simulink model "ASM_Traffic_MultiCore"  (R2026a)
settings: Solver=ode1  StartTime=SIM.tstart.v  StopTime=SIM.tend.v  FixedStep=SIM.StepSize.v
PostLoadFcn:
  | if any(exist('dsrtsu_mdlpostloadfcn', 'file') ~= 0), dsrtsu_mdlpostloadfcn('Execute', bdroot); end
  | try, asm_mdl_postloadfcn(bdroot, 'UpdateModel', 3600); catch, disp(lasterr); end,
InitFcn:
  | , if any(exist('rtifpga_mdlclblib', 'file') ~= 0), rtifpga_mdlclblib('Init', bdroot); end,
  | , if any(exist('dsmpb_private', 'file') ~= 0), dsmpb_private('dsmpb_mdlclblib', 'Init', bdroot); end,
model workspace (MAT data in the model file):
  asmReferencePath = [0 0.01 0.02 0.03 0.04 0.05 0.06 0.07 0.08 0.09 0.1 0.11 ... (350007 elements, 50001x7)]
  roadBounds : Simulink.Parameter (value not decoded)
  safetyAxes : Simulink.Parameter (value not decoded)
undefined symbols (not defined in the file): _to_, a0b2, ASM_BrakeHydraulics_DemoSystems, ASM_VehicleDynamics_DemoSystems, b98103fe8ad365046cd0, BrakeCircuit, controllerConfig, CPT, Crankshaft, DiscIntNeverNeededParam, dsmsi, FinalDriveAssembly, MDL, ModeSignals, mu, Pos_BrakePedal_Maneuver, rad, RefSignals, roadFamilyData, roadFamilyId, s_to_rpm, SIM, SoftECU, Suspension, Tire, Transmission
libraries: ASM_Traffic_lib x135, simulink x98, ASM_Utils_lib x77, ASM_VehicleDynamics_lib x70, ASM_Environment_lib x22, dsmpblib x20, dsmsilib x15, MDLD_Utils_lib x10, ASM_BrakeHydraulics_lib x3, sl_discontinuities x2
(part 3 of 65)

== system ASM_Traffic_MultiCore/AnimationInterface/Fellow_Doors ==
  Environment_Animation : Inport
  Bus Selector1 : BusSelector  OutputSignals=UserSignals_Customized.Fellow1_DoorFL,UserSignals_Customized.Fellow2_DoorFL,UserSignals_Customized.Fellow3_DoorFL,UserSignals_Customized.Fellow4_DoorFL,UserSignals_Customized.Fellow5_DoorFL,UserSignals_Customized.Fellow6_DoorFL,UserSignals_Customized.Fellow7_DoorFL,UserSignals_Customized.Fellow8_DoorFL,UserSignals_Customized.Fellow9_DoorFL,UserSignals_Customized.Fellow10_DoorFL,UserSignals_Customized.Fellow11_DoorFL,UserSignals_Customized.Fellow12_DoorFL,UserSignals_Customized.Fellow13_DoorFL,UserSignals_Customized.Fellow14_DoorFL,UserSignals_Customized.Fellow15_DoorFL,UserSignals_Customized.Fellow16_DoorFL,UserSignals_Customized.Fellow17_DoorFL,UserSignals_Customized.Fellow18_DoorFL,UserSignals_Customized.Fellow19_DoorFL,UserSignals_Customized.Fellow20_DoorFL,UserSignals_Customized.Fellow21_DoorFL,UserSignals_Customized.Fellow22_DoorFL,UserSignals_Customized.Fellow23_DoorFL,UserSignals_Customized.Fellow24_DoorFL,UserSignals_Customized.Fellow25_DoorFL,UserSignals_Customized.Fellow26_DoorFL,UserSignals_Customized.Fellow27_DoorFL,UserSignals_Customized.Fellow28_DoorFL,UserSignals_Customized.Fellow29_DoorFL,UserSignals_Customized.Fellow30_DoorFL  OutputAsBus=on
  Bus Selector2 : BusSelector  OutputSignals=UserSignals_Customized.Fellow1_DoorFR,UserSignals_Customized.Fellow2_DoorFR,UserSignals_Customized.Fellow3_DoorFR,UserSignals_Customized.Fellow4_DoorFR,UserSignals_Customized.Fellow5_DoorFR,UserSignals_Customized.Fellow6_DoorFR,UserSignals_Customized.Fellow7_DoorFR,UserSignals_Customized.Fellow8_DoorFR,UserSignals_Customized.Fellow9_DoorFR,UserSignals_Customized.Fellow10_DoorFR,UserSignals_Customized.Fellow11_DoorFR,UserSignals_Customized.Fellow12_DoorFR,UserSignals_Customized.Fellow13_DoorFR,UserSignals_Customized.Fellow14_DoorFR,UserSignals_Customized.Fellow15_DoorFR,UserSignals_Customized.Fellow16_DoorFR,UserSignals_Customized.Fellow17_DoorFR,UserSignals_Customized.Fellow18_DoorFR,UserSignals_Customized.Fellow19_DoorFR,UserSignals_Customized.Fellow20_DoorFR,UserSignals_Customized.Fellow21_DoorFR,UserSignals_Customized.Fellow22_DoorFR,UserSignals_Customized.Fellow23_DoorFR,UserSignals_Customized.Fellow24_DoorFR,UserSignals_Customized.Fellow25_DoorFR,UserSignals_Customized.Fellow26_DoorFR,UserSignals_Customized.Fellow27_DoorFR,UserSignals_Customized.Fellow28_DoorFR,UserSignals_Customized.Fellow29_DoorFR,UserSignals_Customized.Fellow30_DoorFR  OutputAsBus=on
  Bus Selector3 : BusSelector  OutputSignals=UserSignals_Customized.Fellow1_DoorRL,UserSignals_Customized.Fellow2_DoorRL,UserSignals_Customized.Fellow3_DoorRL,UserSignals_Customized.Fellow4_DoorRL,UserSignals_Customized.Fellow5_DoorRL,UserSignals_Customized.Fellow6_DoorRL,UserSignals_Customized.Fellow7_DoorRL,UserSignals_Customized.Fellow8_DoorRL,UserSignals_Customized.Fellow9_DoorRL,UserSignals_Customized.Fellow10_DoorRL,UserSignals_Customized.Fellow11_DoorRL,UserSignals_Customized.Fellow12_DoorRL,UserSignals_Customized.Fellow13_DoorRL,UserSignals_Customized.Fellow14_DoorRL,UserSignals_Customized.Fellow15_DoorRL,UserSignals_Customized.Fellow16_DoorRL,UserSignals_Customized.Fellow17_DoorRL,UserSignals_Customized.Fellow18_DoorRL,UserSignals_Customized.Fellow19_DoorRL,UserSignals_Customized.Fellow20_DoorRL,UserSignals_Customized.Fellow21_DoorRL,UserSignals_Customized.Fellow22_DoorRL,UserSignals_Customized.Fellow23_DoorRL,UserSignals_Customized.Fellow24_DoorRL,UserSignals_Customized.Fellow25_DoorRL,UserSignals_Customized.Fellow26_DoorRL,UserSignals_Customized.Fellow27_DoorRL,UserSignals_Customized.Fellow28_DoorRL,UserSignals_Customized.Fellow29_DoorRL,UserSignals_Customized.Fellow30_DoorRL  OutputAsBus=on
  Bus Selector4 : BusSelector  OutputSignals=UserSignals_Customized.Fellow1_DoorRR,UserSignals_Customized.Fellow2_DoorRR,UserSignals_Customized.Fellow3_DoorRR,UserSignals_Customized.Fellow4_DoorRR,UserSignals_Customized.Fellow5_DoorRR,UserSignals_Customized.Fellow6_DoorRR,UserSignals_Customized.Fellow7_DoorRR,UserSignals_Customized.Fellow8_DoorRR,UserSignals_Customized.Fellow9_DoorRR,UserSignals_Customized.Fellow10_DoorRR,UserSignals_Customized.Fellow11_DoorRR,UserSignals_Customized.Fellow12_DoorRR,UserSignals_Customized.Fellow13_DoorRR,UserSignals_Customized.Fellow14_DoorRR,UserSignals_Customized.Fellow15_DoorRR,UserSignals_Customized.Fellow16_DoorRR,UserSignals_Customized.Fellow17_DoorRR,UserSignals_Customized.Fellow18_DoorRR,UserSignals_Customized.Fellow19_DoorRR,UserSignals_Customized.Fellow20_DoorRR,UserSignals_Customized.Fellow21_DoorRR,UserSignals_Customized.Fellow22_DoorRR,UserSignals_Customized.Fellow23_DoorRR,UserSignals_Customized.Fellow24_DoorRR,UserSignals_Customized.Fellow25_DoorRR,UserSignals_Customized.Fellow26_DoorRR,UserSignals_Customized.Fellow27_DoorRR,UserSignals_Customized.Fellow28_DoorRR,UserSignals_Customized.Fellow29_DoorRR,UserSignals_Customized.Fellow30_DoorRR  OutputAsBus=on
  Bus Selector5 : BusSelector  OutputSignals=UserSignals_Customized.Fellow1_Hood,UserSignals_Customized.Fellow2_Hood,UserSignals_Customized.Fellow3_Hood,UserSignals_Customized.Fellow4_Hood,UserSignals_Customized.Fellow5_Hood,UserSignals_Customized.Fellow6_Hood,UserSignals_Customized.Fellow7_Hood,UserSignals_Customized.Fellow8_Hood,UserSignals_Customized.Fellow9_Hood,UserSignals_Customized.Fellow10_Hood,UserSignals_Customized.Fellow11_Hood,UserSignals_Customized.Fellow12_Hood,UserSignals_Customized.Fellow13_Hood,UserSignals_Customized.Fellow14_Hood,UserSignals_Customized.Fellow15_Hood,UserSignals_Customized.Fellow16_Hood,UserSignals_Customized.Fellow17_Hood,UserSignals_Customized.Fellow18_Hood,UserSignals_Customized.Fellow19_Hood,UserSignals_Customized.Fellow20_Hood,UserSignals_Customized.Fellow21_Hood,UserSignals_Customized.Fellow22_Hood,UserSignals_Customized.Fellow23_Hood,UserSignals_Customized.Fellow24_Hood,UserSignals_Customized.Fellow25_Hood,UserSignals_Customized.Fellow26_Hood,UserSignals_Customized.Fellow27_Hood,UserSignals_Customized.Fellow28_Hood,UserSignals_Customized.Fellow29_Hood,UserSignals_Customized.Fellow30_Hood  OutputAsBus=on
  Bus Selector6 : BusSelector  OutputSignals=UserSignals_Customized.Fellow1_Trunk,UserSignals_Customized.Fellow2_Trunk,UserSignals_Customized.Fellow3_Trunk,UserSignals_Customized.Fellow4_Trunk,UserSignals_Customized.Fellow5_Trunk,UserSignals_Customized.Fellow6_Trunk,UserSignals_Customized.Fellow7_Trunk,UserSignals_Customized.Fellow8_Trunk,UserSignals_Customized.Fellow9_Trunk,UserSignals_Customized.Fellow10_Trunk,UserSignals_Customized.Fellow11_Trunk,UserSignals_Customized.Fellow12_Trunk,UserSignals_Customized.Fellow13_Trunk,UserSignals_Customized.Fellow14_Trunk,UserSignals_Customized.Fellow15_Trunk,UserSignals_Customized.Fellow16_Trunk,UserSignals_Customized.Fellow17_Trunk,UserSignals_Customized.Fellow18_Trunk,UserSignals_Customized.Fellow19_Trunk,UserSignals_Customized.Fellow20_Trunk,UserSignals_Customized.Fellow21_Trunk,UserSignals_Customized.Fellow22_Trunk,UserSignals_Customized.Fellow23_Trunk,UserSignals_Customized.Fellow24_Trunk,UserSignals_Customized.Fellow25_Trunk,UserSignals_Customized.Fellow26_Trunk,UserSignals_Customized.Fellow27_Trunk,UserSignals_Customized.Fellow28_Trunk,UserSignals_Customized.Fellow29_Trunk,UserSignals_Customized.Fellow30_Trunk  OutputAsBus=on
  Bus to Vector{1..6} (6 alike) : BusToVector
  Data Type Conversion{1..6} (6 alike) : DataTypeConversion  OutDataTypeStr=double  SaturateOnIntegerOverflow=off  RndMeth=Floor
  Multiport Switch : MultiPortSwitch  Inputs=2  OutMin=30  OutMax=30  OutDataTypeStr=double  SaturateOnIntegerOverflow=off
  Multiport Switch{1..5} (5 alike) : MultiPortSwitch  Inputs=2  SaturateOnIntegerOverflow=off  InputSameDT=off
  Mux : Mux  Inputs=6
  Saturation : Saturate  UpperLimit=1  LowerLimit=0
  Select_Signals : Subsystem
  Fellow_Doors : Outport  VectorParamsAs1DForOutWhenUnconnected=off
  wires:
  Saturation/1 -> Fellow_Doors/1
  Environment_Animation/1 -> Select_Signals/1(Fellow_Doors), Bus Selector1/1, Bus Selector3/1, Bus Selector4/1, Bus Selector5/1, Bus Selector6/1, Bus Selector2/1
  Mux/1 -> Saturation/1
  Multiport Switch/1 -> Mux/1
  Multiport Switch1/1 -> Mux/2
  Multiport Switch2/1 -> Mux/3
  Multiport Switch3/1 -> Mux/4
  Multiport Switch5/1 -> Mux/6
  Multiport Switch4/1 -> Mux/5
  Select_Signals/7(SW_Trunk[Open0_1Closed]) -> Multiport Switch5/3
  Select_Signals/6(SW_Hood[Open0_1Closed]) -> Multiport Switch4/3
  Select_Signals/5(SW_DoorRR[Open0_1Closed]) -> Multiport Switch3/3
  Select_Signals/4(SW_DoorRL[Open0_1Closed]) -> Multiport Switch2/3
  Select_Signals/3(SW_DoorFR[Open0_1Closed]) -> Multiport Switch1/3
  Data Type Conversion2/1 -> Multiport Switch1/2
  Data Type Conversion3/1 -> Multiport Switch2/2
  Data Type Conversion4/1 -> Multiport Switch3/2
  Bus Selector6/1 -> Bus to Vector6/1
  Data Type Conversion6/1 -> Multiport Switch5/2
  Bus to Vector6/1 -> Data Type Conversion6/1
  Bus Selector5/1 -> Bus to Vector5/1
  Data Type Conversion5/1 -> Multiport Switch4/2
  Bus to Vector5/1 -> Data Type Conversion5/1
  Bus Selector4/1 -> Bus to Vector4/1
  Bus to Vector4/1 -> Data Type Conversion4/1
  Bus Selector3/1 -> Bus to Vector3/1
  Bus to Vector3/1 -> Data Type Conversion3/1
  Bus Selector2/1 -> Bus to Vector2/1
  Bus to Vector2/1 -> Data Type Conversion2/1
  Data Type Conversion1/1 -> Multiport Switch/2
  Bus to Vector1/1 -> Data Type Conversion1/1
  Bus Selector1/1 -> Bus to Vector1/1
  Select_Signals/2(SW_DoorFL[Open0_1Closed]) -> Multiport Switch/3
  Select_Signals/1(SW_ManualControl_Doors[1Scheduler|2Manual]) -> Multiport Switch/1, Multiport Switch1/1, Multiport Switch2/1, Multiport Switch3/1, Multiport Switch4/1, Multiport Switch5/1

== system ASM_Traffic_MultiCore/AnimationInterface/Fellow_Lights ==
  Environment_Animation : Inport
  Bus Selector : BusSelector  OutputSignals=Fellow1_TurnLights,Fellow2_TurnLights,Fellow3_TurnLights,Fellow4_TurnLights,Fellow5_TurnLights,Fellow6_TurnLights,Fellow7_TurnLights,Fellow8_TurnLights,Fellow9_TurnLights,Fellow10_TurnLights,Fellow11_TurnLights,Fellow12_TurnLights,Fellow13_TurnLights,Fellow14_TurnLights,Fellow15_TurnLights,Fellow16_TurnLights,Fellow17_TurnLights,Fellow18_TurnLights,Fellow19_TurnLights,Fellow20_TurnLights,Fellow21_TurnLights,Fellow22_TurnLights,Fellow23_TurnLights,Fellow24_TurnLights,Fellow25_TurnLights,Fellow26_TurnLights,Fellow27_TurnLights,Fellow28_TurnLights,Fellow29_TurnLights,Fellow30_TurnLights  OutputAsBus=on
  Bus Selector2 : BusSelector  OutputSignals=a_Fellows[m|s2],Settings,UserSignals_Customized
  Bus to Vector3 : BusToVector
  Coding : Subsystem
  Compare_Both : simulink/Logic and Bit Operations/Compare To Constant  relop===  const=3  OutDataTypeStr=boolean
  Compare_Turnlight_L : simulink/Logic and Bit Operations/Compare To Constant  relop===  const=1  OutDataTypeStr=boolean
  Compare_Turnlight_R : simulink/Logic and Bit Operations/Compare To Constant  relop===  const=2  OutDataTypeStr=boolean
  Gain : Gain  Gain=-1
  Multiport Switch : MultiPortSwitch  Inputs=2  SaturateOnIntegerOverflow=off  InputSameDT=off
  Multiport Switch4 : MultiPortSwitch  Inputs=2  SaturateOnIntegerOverflow=off  InputSameDT=off
  Mux : Mux  Inputs=3
  OR : Logic  Operator=OR  IconShape=distinctive  AllPortsSameDT=off  OutDataTypeStr=boolean
  OR1 : Logic  Operator=OR  IconShape=distinctive  AllPortsSameDT=off  OutDataTypeStr=boolean
  Relay : Relay  OnSwitchValue=1.3  OffSwitchValue=1.2  OutDataTypeStr=boolean
  Select_Signals : Subsystem
  TurnLights[0|1|2|3] : DataTypeConversion  OutDataTypeStr=uint32  SaturateOnIntegerOverflow=off  RndMeth=Floor
  Fellow_Light : Outport  VectorParamsAs1DForOutWhenUnconnected=off
  wires:
  Gain/1 -> Relay/1
  Bus Selector2/2 -> Select_Signals/1(Fellow_VehicleLights)  "<Settings>"
  Environment_Animation/1 -> Bus Selector2/1
  Select_Signals/3(SW_TurnLight[0Off|1Left|2Right|3Both]) -> Multiport Switch4/3
  Select_Signals/2(SW_BrakeLight[0Off|1On]) -> Multiport Switch/3
  Select_Signals/1(SW_ManualControl_Lights[1Scheduler|2Manual]) -> Multiport Switch/1, Multiport Switch4/1
  Bus to Vector3/1 -> TurnLights[0|1|2|3]/1
  Mux/1 -> Coding/1(FellowLights)
  Multiport Switch4/1 -> Compare_Both/1, Compare_Turnlight_R/1, Compare_Turnlight_L/1
  OR1/1 -> Mux/3
  OR/1 -> Mux/2
  Compare_Both/1 -> OR/2, OR1/2
  Multiport Switch/1 -> Mux/1
  Compare_Turnlight_R/1 -> OR1/1
  Compare_Turnlight_L/1 -> OR/1
  Relay/1 -> Multiport Switch/2
  TurnLights[0|1|2|3]/1 -> Multiport Switch4/2
  Coding/1(Out) -> Fellow_Light/1
  Bus Selector2/1 -> Gain/1  "<a_Fellows[m|s2]>"
  Bus Selector2/3 -> Bus Selector/1  "<UserSignals_Customized>"
  Bus Selector/1 -> Bus to Vector3/1

== system ASM_Traffic_MultiCore/AnimationInterface/OpenAnimationInterfaceModel ==

== system ASM_Traffic_MultiCore/AnimationInterface/Vehicle_Doors ==
  Environment_Animation : Inport
  Bus Selector : BusSelector  OutputSignals=Mnv_DoorFL[],Mnv_DoorFR[],Mnv_DoorRL[],Mnv_DoorRR[],Mnv_Hood[],Mnv_Trunk[]  OutputAsBus=on
  Bus Selector7 : BusSelector  OutputSignals=Sw_ManualControl_Doors[1Maneuver|2Manual]
  Bus Selector8 : BusSelector  OutputSignals=Sw_DoorFL[0Closed_1Open],Sw_DoorFR[0Closed_1Open],Sw_DoorRL[0Closed_1Open],Sw_DoorRR[0Closed_1Open],Sw_Hood[0Closed_1Open],Sw_Trunk[0Closed_1Open]  OutputAsBus=on
  Bus to Vector : BusToVector
  Bus to Vector7 : BusToVector
  Data Type Conversion : DataTypeConversion  OutDataTypeStr=double  SaturateOnIntegerOverflow=off  RndMeth=Floor
  Data Type Conversion7 : DataTypeConversion  OutDataTypeStr=uint32  SaturateOnIntegerOverflow=off  RndMeth=Floor
  Data Type Conversion8 : DataTypeConversion  OutDataTypeStr=double  SaturateOnIntegerOverflow=off  RndMeth=Floor
  Multiport Switch6 : MultiPortSwitch  Inputs=2  OutMin=30  OutMax=30  OutDataTypeStr=double  SaturateOnIntegerOverflow=off
  Saturation : Saturate  UpperLimit=1  LowerLimit=0
  ASM_Vehicle_Doors : Outport  VectorParamsAs1DForOutWhenUnconnected=off
  wires:
  Saturation/1 -> ASM_Vehicle_Doors/1
  Data Type Conversion7/1 -> Multiport Switch6/1
  Bus Selector7/1 -> Data Type Conversion7/1  "<Sw_ManualControl_Doors[1Maneuver|2Manual]>"
  Data Type Conversion8/1 -> Multiport Switch6/3
  Multiport Switch6/1 -> Saturation/1
  Bus to Vector7/1 -> Data Type Conversion8/1
  Bus to Vector/1 -> Data Type Conversion/1
  Bus Selector8/1 -> Bus to Vector7/1
  Data Type Conversion/1 -> Multiport Switch6/2
  Environment_Animation/1 -> Bus Selector/1, Bus Selector7/1, Bus Selector8/1
  Bus Selector/1 -> Bus to Vector/1

== system ASM_Traffic_MultiCore/AnimationInterface/Vehicle_Lights ==
  VehicleDynamics_Animation : Inport
  Environment_Animation : Inport  Port=2
  Bus Selector : BusSelector  OutputSignals=Sw_ManualControl_Lights[1Maneuver|2Manual],Sw_BrakeLight[0Off|1On],Sw_TurnLights[0Off|1Left|2Right|3Both],ASM_Vehicle_TurnLights[]
  Bus Selector13 : BusSelector  OutputSignals=p_Brake[FL;FR;RL;RR][bar]
  Cmp_BrakePres : simulink/Logic and Bit Operations/Compare To Constant  relop=>  const=3  OutDataTypeStr=boolean
  Coding : Subsystem
  Compare_Hazard : simulink/Logic and Bit Operations/Compare To Constant  relop===  const=3  OutDataTypeStr=boolean
  Compare_Turnlight_L : simulink/Logic and Bit Operations/Compare To Constant  relop===  const=1.0  OutDataTypeStr=boolean
  Compare_Turnlight_R : simulink/Logic and Bit Operations/Compare To Constant  relop===  const=2  OutDataTypeStr=boolean
  Data Type Conversion1 : DataTypeConversion  OutDataTypeStr=boolean  SaturateOnIntegerOverflow=off  RndMeth=Floor
  Data Type Conversion2 : DataTypeConversion  OutDataTypeStr=uint32  SaturateOnIntegerOverflow=off  RndMeth=Floor
  Data Type Conversion3 : DataTypeConversion  OutDataTypeStr=uint32  SaturateOnIntegerOverflow=off  RndMeth=Floor
  Data Type Conversion4 : DataTypeConversion  OutDataTypeStr=uint32  SaturateOnIntegerOverflow=off  RndMeth=Floor
  Gain : Gain  Gain=1/4
  Multiport Switch : MultiPortSwitch  Inputs=2  SaturateOnIntegerOverflow=off  InputSameDT=off
  Multiport Switch4 : MultiPortSwitch  Inputs=2  SaturateOnIntegerOverflow=off  InputSameDT=off
  Mux : Mux  Inputs=3
  OR : Logic  Operator=OR  IconShape=distinctive  AllPortsSameDT=off  OutDataTypeStr=boolean
  OR1 : Logic  Operator=OR  IconShape=distinctive  AllPortsSameDT=off  OutDataTypeStr=boolean
  Sum of Elements : Sum  Inputs=+
  ASM_Vehicle_Lights : Outport  VectorParamsAs1DForOutWhenUnconnected=off
  wires:
  Bus Selector13/1 -> Sum of Elements/1  "<p_Brake[FL;FR;RL;RR][bar]>"
  Compare_Turnlight_L/1 -> OR/1
  Gain/1 -> Cmp_BrakePres/1
  Multiport Switch/1 -> Mux/1
  Data Type Conversion3/1 -> Multiport Switch/1, Multiport Switch4/1
  Compare_Hazard/1 -> OR/2, OR1/2
  Bus Selector/1 -> Data Type Conversion3/1  "<Sw_ManualControl_Lights[1Maneuver|2Manual]>"
  Bus Selector/3 -> Data Type Conversion2/1  "<Sw_TurnLights[0Off|1Left|2Right|3Both]>"
  Data Type Conversion4/1 -> Multiport Switch4/2
  Sum of Elements/1 -> Gain/1
  Bus Selector/4 -> Data Type Conversion4/1  "<ASM_Vehicle_TurnLights[]>"
  Bus Selector/2 -> Data Type Conversion1/1  "<Sw_BrakeLight[0Off|1On]>"
  Compare_Turnlight_R/1 -> OR1/1
  OR1/1 -> Mux/3
  Cmp_BrakePres/1 -> Multiport Switch/2
  Data Type Conversion2/1 -> Multiport Switch4/3
  OR/1 -> Mux/2
  Data Type Conversion1/1 -> Multiport Switch/3
  Multiport Switch4/1 -> Compare_Hazard/1, Compare_Turnlight_R/1, Compare_Turnlight_L/1
  Mux/1 -> Coding/1(In)
  Coding/1(Out) -> ASM_Vehicle_Lights/1
  Environment_Animation/1 -> Bus Selector/1
  VehicleDynamics_Animation/1 -> Bus Selector13/1

== system ASM_Traffic_MultiCore/DomainControl/DriverAssistance ==
  note: Driver Assistance
  In : Inport
  Control : Subsystem
  Interface_In : Subsystem
  Interface_Out : Subsystem
  SignalInterface : Subsystem
  Out : Outport  VectorParamsAs1DForOutWhenUnconnected=off
  wires:
  In/1 -> Interface_In/1(In)
  Interface_In/1(Out) -> SignalInterface/1(In), Control/1(Interface_In)
  Interface_Out/1(Out) -> Out/1
  Control/1(Control) -> Interface_Out/1(In)

== system ASM_Traffic_MultiCore/DomainControl/StartSystem ==
  note: Start System
  In : Inport
  Control : Subsystem
  Interface_In : Subsystem
  Interface_Out : Subsystem
  SignalInterface : Subsystem
  Out : Outport  VectorParamsAs1DForOutWhenUnconnected=off
  wires:
  In/1 -> Interface_In/1(In)
  Interface_In/1(Out) -> SignalInterface/1(In), Control/1(Interface_In)
  Interface_Out/1(Out) -> Out/1
  Control/1(Control) -> Interface_Out/1(In)

== system ASM_Traffic_MultiCore/DomainControl/TorqueManager ==
  note: Torque Manager Basic
  In : Inport
  Control : Subsystem
  Interface_In : Subsystem
  Interface_Out : Subsystem
  SignalInterface : Subsystem
  Out : Outport  VectorParamsAs1DForOutWhenUnconnected=off
  wires:
  In/1 -> Interface_In/1(In)
  Control/1(Control) -> Interface_Out/1(In)
  Interface_In/1(Out) -> SignalInterface/1(In), Control/1(Interface_In)
  Interface_Out/1(Out) -> Out/1

== system ASM_Traffic_MultiCore/Driver/Interface_In ==
  note: Driver
  In : Inport
  Bus Creator1 : BusCreator  Inputs=1
  Bus Selector4 : BusSelector  OutputSignals=Environment.Plant.Sw_ModelPortBlocks[0Disabled|1Enabled],Environment.Plant.Sw_ModelDeskPlottingInterface[0Disabled|1Enabled],VehicleDynamics.Plant.v_x_Vehicle_CoG[km|h],VehicleDynamics.Plant.v_y_Vehicle_CoG[km|h],VehicleDynamics.Plant.Pos_x_Vehicle_CoorSys_E[m],VehicleDynamics.Plant.Pos_y_Vehicle_CoorSys_E[m],VehicleDynamics.Plant.Angle_Yaw_Vehicle_CoorSys_E[deg],VehicleDynamics.Plant.YawRate_Vehicle_CoG[deg|s],VehicleDynamics.Plant.m_TotalVehicle[kg],VehicleDynamics.Plant.F_Driving_Res[N],VehicleDynamics.Plant.Pos_x_CoG_Vehicle_Total[m],VehicleDynamics.Plant.Inertia_z_Vehicle_Total[kgm2],VehicleDynamics.Plant.CorneringStiffness_Tire_Front[N|rad],VehicleDynamics.Plant.CorneringStiffness_Tire_Rear[N|rad],VehicleDynamics.Plant.i_Steering_Mean[],Drivetrain.Plant.n_Engine[rpm],Drivetrain.Plant.omega_Out_Trm[rad|s],DomainControl.TorqueManager.Control.State_Engine[0|1|2|3|4],Environment.Plant.Reset_States[0|1],Environment.Plant.s_Vehicle_Init[m],Environment.Plant.Route_Direction_Init[],Environment.Plant.s_Total_Vehicle_Road[m],Environment.Plant.Curv_Preview_Road[1|m],Environment.Plant.Speed_Limit_Preview_Road[km|h],Environment.Plant.Pos_z_Preview_Road[m],Environment.Plant.Roll_Preview_Road[deg],Environment.Plant.Pitch_Preview_Road[deg],Environment.Plant.x_Preview_DriverCurv[m],Environment.Plant.y_Preview_DriverCurv[m],Environment.Plant.Pos_x_Preview_Road[m],Environment.Plant.Pos_y_Preview_Road[m],Environment.Plant.Dist_Border_Left[m],Environment.Plant.Dist_Border_Right[m],Environment.Plant.Curv_Vehicle_Road[1|m],Environment.Plant.Angle_Yaw_Veh_Road[deg],Environment.Plant.Pos_AccPedal_Maneuver[%],Environment.Plant.Pos_BrakePedal_Maneuver[%],Environment.Plant.Pos_ClutchPedal_Maneuver[%],Environment.Plant.Gear_Maneuver[],Environment.Plant.Angle_SteeringWheel_Maneuver[deg],Environment.Plant.SelectorLever_Maneuver[-3T|-2P|-1R|0N|1D],Environment.Plant.v_Vehicle_Ref_Maneuver[m|s],Environment.Plant.v_Vehicle_Preview_Ref_Maneuver[m|s],Environment.Plant.a_x_Max[m|s2],Environment.Plant.a_x_Min[m|s2],Environment.Plant.a_y_Max[m|s2],Environment.Plant.Gear_Max[0Off|1_n],Environment.Plant.a_x_Vehicle_Ref_TrafficDriver[m|s2],Environment.Plant.Width_Deadzone_LatCtrl[m],Environment.Plant.Pos_x_Ref_Vehicle_Road[m],Environment.Plant.Pos_y_Ref_Vehicle_Road[m],Environment.Plant.Enable_v_Init[0|1],Drivetrain.Plant.Mode_Transmission[1Manual|2Automatic],Environment.Plant.Mode_AcceleratorBrake[1Stim|2Driver],Environment.Plant.Mode_GearClutch[1Stim|2Driver|3OpenClutch|4RefGear],Environment.Plant.Mode_Steer[1Stim|2Driver|3Fix],Environment.Plant.Sw_LatDriver[1LatCtrl1|2LatCtrl2],Environment.Plant.Mode_LatCtrl[1Pos|2Yaw],Environment.Plant.Mode_AdaptVelocityToRoad[1Off|2On],Environment.Plant.Mode_ForceToRoad[1Off|2On],Environment.Plant.Mode_SelectorLever[1Stim|2Driver],Environment.Plant.Mode_CurvatureCalculation[1Road|2Driver],Environment.Plant.Mode_TrafficDriver[1Off|2On],Engine.Control.State_StartStop[1Off|2NotReady|3Ready|4EngStopped],Engine.Control.n_Engine_Idle_Set[rpm],Environment.Plant.Lane_ID_Vehicle[]
  ModelSignals : Subsystem
  Out : Outport  VectorParamsAs1DForOutWhenUnconnected=off
  wires:
  Bus Selector4/2 -> ModelSignals/2(Sw_ModelDeskPlottingInterface[0Disabled|1Enabled])  "<Sw_ModelDeskPlottingInterface[0Disabled|1Enabled]>"
  Bus Selector4/1 -> ModelSignals/1(Sw_ModelPortBlocks[0Disabled|1Enabled])  "<Sw_ModelPortBlocks[0Disabled|1Enabled]>"
  In/1 -> Bus Selector4/1
  Bus Selector4/51 -> ModelSignals/51(Pos_y_Ref_Vehicle_Road[m])  "<Pos_y_Ref_Vehicle_Road[m]>"
  Bus Selector4/50 -> ModelSignals/50(Pos_x_Ref_Vehicle_Road[m])  "<Pos_x_Ref_Vehicle_Road[m]>"
  Bus Selector4/49 -> ModelSignals/49(Width_Deadzone_LatCtrl[m])  "<Width_Deadzone_LatCtrl[m]>"
  Bus Selector4/48 -> ModelSignals/48(a_x_Vehicle_Ref_TrafficDriver[m|s2])  "<a_x_Vehicle_Ref_TrafficDriver[m|s2]>"
  Bus Selector4/47 -> ModelSignals/47(Gear_Max[0Off|1_n])  "<Gear_Max[0Off|1_n]>"
  Bus Selector4/46 -> ModelSignals/46(a_y_Max[m|s2])  "<a_y_Max[m|s2]>"
  Bus Selector4/45 -> ModelSignals/45(a_x_Min[m|s2])  "<a_x_Min[m|s2]>"
  Bus Selector4/44 -> ModelSignals/44(a_x_Max[m|s2])  "<a_x_Max[m|s2]>"
  Bus Selector4/43 -> ModelSignals/43(v_Vehicle_Preview_Ref_Maneuver[m|s])  "<v_Vehicle_Preview_Ref_Maneuver[m|s]>"
  Bus Selector4/42 -> ModelSignals/42(v_Vehicle_Ref_Maneuver[m|s])  "<v_Vehicle_Ref_Maneuver[m|s]>"
  Bus Selector4/41 -> ModelSignals/41(SelectorLever_Maneuver[-3T|-2P|-1R|0N|1D])  "<SelectorLever_Maneuver[-3T|-2P|-1R|0N|1D]>"
  Bus Selector4/40 -> ModelSignals/40(Angle_SteeringWheel_Maneuver[deg])  "<Angle_SteeringWheel_Maneuver[deg]>"
  Bus Selector4/39 -> ModelSignals/39(Gear_Maneuver[])  "<Gear_Maneuver[]>"
  Bus Selector4/38 -> ModelSignals/38(Pos_ClutchPedal_Maneuver[%])  "<Pos_ClutchPedal_Maneuver[%]>"
  Bus Selector4/37 -> ModelSignals/37(Pos_BrakePedal_Maneuver[%])  "<Pos_BrakePedal_Maneuver[%]>"
  Bus Selector4/36 -> ModelSignals/36(Pos_AccPedal_Maneuver[%])  "<Pos_AccPedal_Maneuver[%]>"
  Bus Selector4/35 -> ModelSignals/35(Angle_Yaw_Veh_Road[deg])  "<Angle_Yaw_Veh_Road[deg]>"
  Bus Selector4/34 -> ModelSignals/34(Curv_Veh_Road[1|m])  "<Curv_Vehicle_Road[1|m]>"
  Bus Selector4/33 -> ModelSignals/33(Dist_Border_Right[m])  "<Dist_Border_Right[m]>"
  Bus Selector4/32 -> ModelSignals/32(Dist_Border_Left[m])  "<Dist_Border_Left[m]>"
  Bus Selector4/31 -> ModelSignals/31(Pos_y_Preview_Road[m])  "<Pos_y_Preview_Road[m]>"
  Bus Selector4/30 -> ModelSignals/30(Pos_x_Preview_Road[m])  "<Pos_x_Preview_Road[m]>"
  Bus Selector4/29 -> ModelSignals/29(Pos_y_Preview_DriverCurv[m])  "<y_Preview_DriverCurv[m]>"
  Bus Selector4/28 -> ModelSignals/28(Pos_x_Preview_DriverCurv[m])  "<x_Preview_DriverCurv[m]>"
  Bus Selector4/27 -> ModelSignals/27(Pitch_Preview_Road[deg])  "<Pitch_Preview_Road[deg]>"
  Bus Selector4/26 -> ModelSignals/26(Roll_Preview_Road[deg])  "<Roll_Preview_Road[deg]>"
  Bus Selector4/25 -> ModelSignals/25(Pos_z_Preview_Road[m])  "<Pos_z_Preview_Road[m]>"
  Bus Selector4/24 -> ModelSignals/24(Speed_Limit_Preview_Road[km|h])  "<Speed_Limit_Preview_Road[km|h]>"
  Bus Selector4/23 -> ModelSignals/23(Curv_Preview_Road[1|m])  "<Curv_Preview_Road[1|m]>"
  Bus Selector4/22 -> ModelSignals/22(s_Total_Vehicle_Road[m])  "<s_Total_Vehicle_Road[m]>"
  Bus Selector4/21 -> ModelSignals/21(Route_Direction_Init[])  "<Route_Direction_Init[]>"
  Bus Selector4/20 -> ModelSignals/20(s_Vehicle_Init[m])  "<s_Vehicle_Init[m]>"
  Bus Selector4/19 -> ModelSignals/19(Reset_States[0|1])  "<Reset_States[0|1]>"
  Bus Creator1/1 -> Out/1
  Bus Selector4/52 -> ModelSignals/52(Enable_v_Init[0|1])  "<Enable_v_Init[0|1]>"
  Bus Selector4/53 -> ModelSignals/53(Mode_Transmission[1Manual|2Automatic])  "<Mode_Transmission[1Manual|2Automatic]>"
  Bus Selector4/54 -> ModelSignals/54(Mode_AcceleratorBrake[1Stim|2Driver])  "<Mode_AcceleratorBrake[1Stim|2Driver]>"
  Bus Selector4/55 -> ModelSignals/55(Mode_GearClutch[1Stim|2Driver|3OpenClutch|4RefGear])  "<Mode_GearClutch[1Stim|2Driver|3OpenClutch|4RefGear]>"
  Bus Selector4/56 -> ModelSignals/56(Mode_Steer[1Stim|2Driver|3Fix])  "<Mode_Steer[1Stim|2Driver|3Fix]>"
  Bus Selector4/57 -> ModelSignals/57(Sw_LatDriver[1LatCtrl1|2LatCtrl2])  "<Sw_LatDriver[1LatCtrl1|2LatCtrl2]>"
  Bus Selector4/58 -> ModelSignals/58(Mode_LatCtrl[1Pos|2Yaw])  "<Mode_LatCtrl[1Pos|2Yaw]>"
  Bus Selector4/59 -> ModelSignals/59(Mode_AdaptVelocityToRoad[1Off|2On])  "<Mode_AdaptVelocityToRoad[1Off|2On]>"
  Bus Selector4/60 -> ModelSignals/60(Mode_ForceToRoad[1Off|2On])  "<Mode_ForceToRoad[1Off|2On]>"
  Bus Selector4/61 -> ModelSignals/61(Mode_SelectorLever[1Stim|2Driver])  "<Mode_SelectorLever[1Stim|2Driver]>"
  Bus Selector4/62 -> ModelSignals/62(Mode_CurvatureCalculation[1Road|2Driver])  "<Mode_CurvatureCalculation[1Road|2Driver]>"
  Bus Selector4/63 -> ModelSignals/63(Mode_TrafficDriver[1Off|2On])  "<Mode_TrafficDriver[1Off|2On]>"
  Bus Selector4/65 -> ModelSignals/65(n_Engine_Idle_Set[rpm])  "<n_Engine_Idle_Set[rpm]>"
  Bus Selector4/64 -> ModelSignals/64(State_StartStop[1Off|2NotReady|3Ready|4EngStopped])  "<State_StartStop[1Off|2NotReady|3Ready|4EngStopped]>"
  Bus Selector4/18 -> ModelSignals/18(State_Engine[0|1|2|3|4])  "<State_Engine[0|1|2|3|4]>"
  Bus Selector4/17 -> ModelSignals/17(omega_Out_Trm[rad|s])  "<omega_Out_Trm[rad|s]>"
  Bus Selector4/16 -> ModelSignals/16(n_Engine[rpm])  "<n_Engine[rpm]>"
  Bus Selector4/15 -> ModelSignals/15(i_Steering_Mean[])  "<i_Steering_Mean[]>"
  Bus Selector4/14 -> ModelSignals/14(CorneringStiffness_Tire_Rear[N|rad])  "<CorneringStiffness_Tire_Rear[N|rad]>"
  Bus Selector4/13 -> ModelSignals/13(CorneringStiffness_Tire_Front[N|rad])  "<CorneringStiffness_Tire_Front[N|rad]>"
  Bus Selector4/12 -> ModelSignals/12(Inertia_z_Vehicle_Total[kgm2])  "<Inertia_z_Vehicle_Total[kgm2]>"
  Bus Selector4/11 -> ModelSignals/11(Pos_x_CoG_Vehicle_Total[m])  "<Pos_x_CoG_Vehicle_Total[m]>"
  Bus Selector4/10 -> ModelSignals/10(F_Driving_Res[N])  "<F_Driving_Res[N]>"
  Bus Selector4/9 -> ModelSignals/9(m_Total_Vehicle[kg])  "<m_TotalVehicle[kg]>"
  Bus Selector4/8 -> ModelSignals/8(YawRate_Vehicle[deg|s])  "<YawRate_Vehicle_CoG[deg|s]>"
  Bus Selector4/7 -> ModelSignals/7(Angle_Yaw_Vehicle_CoorSys_E[deg])  "<Angle_Yaw_Vehicle_CoorSys_E[deg]>"
  Bus Selector4/6 -> ModelSignals/6(Pos_y_Vehicle_CoorSys_E[m])  "<Pos_y_Vehicle_CoorSys_E[m]>"
  Bus Selector4/5 -> ModelSignals/5(Pos_x_Vehicle_CoorSys_E[m])  "<Pos_x_Vehicle_CoorSys_E[m]>"
  Bus Selector4/4 -> ModelSignals/4(v_y_Vehicle_CoG[km|h])  "<v_y_Vehicle_CoG[km|h]>"
  Bus Selector4/3 -> ModelSignals/3(v_x_Vehicle_CoG[km|h])  "<v_x_Vehicle_CoG[km|h]>"
  ModelSignals/1(Out) -> Bus Creator1/1
  Bus Selector4/66 -> ModelSignals/66(Lane_ID_Vehicle[])  "<Lane_ID_Vehicle[]>"

== system ASM_Traffic_MultiCore/Driver/Interface_Out ==
  note: Driver
  In : Inport
  Bus Creator1 : BusCreator  Inputs=1
  Bus Selector2 : BusSelector  OutputSignals=OutputSignals.Pos_AccPedal[%],OutputSignals.Pos_BrakePedal[%],OutputSignals.Pos_ClutchPedal[%],OutputSignals.Gear[],OutputSignals.SelectorLever[-3T|-2P|-1R|0N|1D],OutputSignals.s_Preview[m],OutputSignals.Angle_SteeringWheel[deg],LongitudinalController.LongCtrl.t_Preview[s]
  Plant_ModelSignals : Subsystem
  Out : Outport  VectorParamsAs1DForOutWhenUnconnected=off
  wires:
  Bus Selector2/6 -> Plant_ModelSignals/6(s_Preview[m])  "<s_Preview[m]>"
  Bus Selector2/8 -> Plant_ModelSignals/8(t_Preview_vRef_Driver[s])  "<t_Preview[s]>"
  Bus Selector2/5 -> Plant_ModelSignals/5(SelectorLever[-3T|-2P|-1R|0N|1D])  "<SelectorLever[-3T|-2P|-1R|0N|1D]>"
  Bus Selector2/4 -> Plant_ModelSignals/4(Gear[])  "<Gear[]>"
  Bus Selector2/3 -> Plant_ModelSignals/3(Pos_ClutchPedal[%])  "<Pos_ClutchPedal[%]>"
  Bus Selector2/2 -> Plant_ModelSignals/2(Pos_BrakePedal[%])  "<Pos_BrakePedal[%]>"
  Bus Selector2/1 -> Plant_ModelSignals/1(Pos_AccPedal[%])  "<Pos_AccPedal[%]>"
  In/1 -> Bus Selector2/1
  Bus Selector2/7 -> Plant_ModelSignals/7(Angle_SteeringWheel[deg])  "<Angle_SteeringWheel[deg]>"
  Bus Creator1/1 -> Out/1  "Driver"
  Plant_ModelSignals/1(Out) -> Bus Creator1/1

== system ASM_Traffic_MultiCore/Driver/Plant ==
  note: Driver
  Interface_In : Inport
  steering_wheel[deg] : Inport  Port=2
  Driver : Subsystem
  UserInterface : Subsystem
  Plant : Outport  VectorParamsAs1DForOutWhenUnconnected=off
  wires:
  Driver/1(ASMSignalBus) -> Plant/1, UserInterface/1(In)
  Interface_In/1 -> Driver/2(Interface_In), UserInterface/2(Interface_In)
  UserInterface/1(Out) -> Driver/1(UserInterface)
  steering_wheel[deg]/1 -> Driver/3(steering_wheel[deg])

== system ASM_Traffic_MultiCore/Driver/SignalInterface ==
  In : Inport
  ASMSignalInterface : Subsystem  mask(ASM_SIGNAL_INTERFACE){LabelTextfield=Driver}
      mask prompts: LabelTextfield "Label"
      mask help:
      | The ASMSignalInterface block processes the ASMSignalBus and provides a vector-based interface for each signal (e.g. ModelDesk Plotting).
      |
      | Always push the update button after you have changed the signal bus structure in order to synchronize the signal interface. The update may take a few seconds.
      | A modified model must be reloaded in ModelDesk to keep consistency of ModelDesk and simulation model plot signals. Therefore select ''Update Model'' from the ''Simulation Model'' context menu of the ModelDesk Project Navigator.
      settings: AttributesFormatString=Label: %<LabelTextfield>
      settings: CopyFcn=|
      | try
      |  set_param(gcb,'LinkStatus', 'none')
      | catch
      | end
      mask Help: eval(['asm_modelhelp(gcbh,''tool'',''ASM_Utils_lib'', ''ASMSIGNALINTERFACE'')'])
      mask DialogControl Hint Prompt: For changes of Label first apply change and then push "Update".
      mask DialogControl UpdateButton Prompt: Update
      mask DialogControl UpdateButton Callback: asm_mdld_plot_block_update(bdroot(gcb), 'update', 'current');
      mask DialogControl UpdateAllButton Prompt: Update All
      mask DialogControl UpdateAllButton Callback: asm_mdld_plot_block_update(bdroot(gcb), 'update', 'all');
  Bus Selector Disable Signals : BusSelector  OutputSignals=ExternalModel.Sw_ModelPortBlocks[0Disabled|1Enabled],ExternalModel.Sw_ModelDeskPlottingInterface[0Disabled|1Enabled]
  ExternalOutports : Subsystem  TreatAsAtomicUnit=on
  wires:
  Bus Selector Disable Signals/2 -> ASMSignalInterface/Enable  "<Sw_ModelDeskPlottingInterface[0Disabled|1Enabled]>"
  Bus Selector Disable Signals/1 -> ExternalOutports/Enable  "<Sw_ModelPortBlocks[0Disabled|1Enabled]>"
  In/1 -> Bus Selector Disable Signals/1
  [ASMBUS_Driver_Plant] -> ASMSignalInterface/1(ASMSignalBus), ExternalOutports/1(In1)

== system ASM_Traffic_MultiCore/Drivetrain/Control ==
  note: Drivetrain Control
  Interface_In : Inport
  Plant : Inport  Port=2
  SoftECU_Drivetrain : Subsystem
  Sw_ECU_Signals : Subsystem
  UserInterface : Subsystem
  Control : Outport  VectorParamsAs1DForOutWhenUnconnected=off
  wires:
  Interface_In/1 -> SoftECU_Drivetrain/2(Interface_In), Sw_ECU_Signals/2(ExternalECU)
  SoftECU_Drivetrain/2(Out) -> Sw_ECU_Signals/1(SoftECU)
  Sw_ECU_Signals/1(ECU_Signals) -> Control/1
  SoftECU_Drivetrain/1(ASMSignalBus) -> UserInterface/1(In)
  UserInterface/1(Out) -> SoftECU_Drivetrain/1(UserInterface)
  Plant/1 -> SoftECU_Drivetrain/3(Plant)

== system ASM_Traffic_MultiCore/Drivetrain/Interface_In ==
  note: Drivetrain
  In : Inport
  Bus Creator1 : BusCreator  Inputs=2
  Bus Selector5 : BusSelector  OutputSignals=Environment.Plant.Sw_ModelPortBlocks[0Disabled|1Enabled],Environment.Plant.Sw_ModelDeskPlottingInterface[0Disabled|1Enabled],Environment.Plant.n_Engine_Set[rpm],Environment.Plant.Sw_Testbench[0Off|1On],Driver.Plant.Pos_ClutchPedal[%],Driver.Plant.Gear[],Environment.Plant.Reset_States[0|1],Engine.Plant.Trq_MeanEff_Engine[Nm],VehicleDynamics.Plant.omega_Wheel[FL;FR;RL;RR][rad|s],Environment.Plant.Enable_v_Init[0|1],Driver.Plant.Pos_AccPedal[%],Driver.Plant.SelectorLever[-3T|-2P|-1R|0N|1D],Environment.Plant.Sw_TipShift_Maneuver[-1Down|0Off|1Up],Environment.Plant.Gear_Maneuver[],Environment.Plant.Mode_GearClutch[1Stim|2Driver|3OpenClutch|4RefGear],Environment.Plant.Gear_Max[0Off|1_n],DomainControl.TorqueManager.Control.State_Engine[0|1|2|3|4],Engine.Control.State_StartStop[1Off|2NotReady|3Ready|4EngStopped],Engine.Control.Sw_Starter[0Off|1On],Engine.Control.CrankAngle_Cyl[aTDC],Engine.Plant.Type_Engine[0Unkown|1Other|2Otto|3Diesel|4Electric]
  Bus Selector51 : BusSelector  OutputSignals=Environment.Plant.Sw_ModelPortBlocks[0Disabled|1Enabled]
  ExternalSignals : Subsystem
  ModelSignals : Subsystem
  Out : Outport  VectorParamsAs1DForOutWhenUnconnected=off
  wires:
  Bus Selector51/1 -> ExternalSignals/Enable  "<Sw_ModelPortBlocks[0Disabled|1Enabled]>"
  ExternalSignals/1(ExternalECU_Transmission_Out) -> Bus Creator1/2
  Bus Selector5/2 -> ModelSignals/2(Sw_ModelDeskPlottingInterface[0Disabled|1Enabled])  "<Sw_ModelDeskPlottingInterface[0Disabled|1Enabled]>"
  Bus Selector5/1 -> ModelSignals/1(Sw_ModelPortBlocks[0Disabled|1Enabled])  "<Sw_ModelPortBlocks[0Disabled|1Enabled]>"
  In/1 -> Bus Selector51/1, Bus Selector5/1
  Bus Creator1/1 -> Out/1
  Bus Selector5/3 -> ModelSignals/3(n_Engine_Set[rpm])  "<n_Engine_Set[rpm]>"
  Bus Selector5/4 -> ModelSignals/4(Sw_Testbench[0Off|1On])  "<Sw_Testbench[0Off|1On]>"
  Bus Selector5/5 -> ModelSignals/5(Pos_ClutchPedal[%])  "<Pos_ClutchPedal[%]>"
  Bus Selector5/6 -> ModelSignals/6(Gear[])  "<Gear[]>"
  Bus Selector5/7 -> ModelSignals/7(Reset_States[0|1])  "<Reset_States[0|1]>"
  Bus Selector5/9 -> ModelSignals/9(omega_Wheel[FL;FR;RL;RR][rad|s])  "<omega_Wheel[FL;FR;RL;RR][rad|s]>"
  Bus Selector5/8 -> ModelSignals/8(Trq_MeanEff_Engine[Nm])  "<Trq_MeanEff_Engine[Nm]>"
  Bus Selector5/10 -> ModelSignals/10(Enable_v_Init[0|1])  "<Enable_v_Init[0|1]>"
  Bus Selector5/11 -> ModelSignals/11(Pos_AccPedal[%])  "<Pos_AccPedal[%]>"
  Bus Selector5/12 -> ModelSignals/12(SelectorLever[-3T|-2P|-1R|0N|1D])  "<SelectorLever[-3T|-2P|-1R|0N|1D]>"
  Bus Selector5/13 -> ModelSignals/13(Sw_TipShift[-1Down|0Off|1Up])  "<Sw_TipShift_Maneuver[-1Down|0Off|1Up]>"
  Bus Selector5/14 -> ModelSignals/14(Gear_Maneuver[])  "<Gear_Maneuver[]>"
  Bus Selector5/15 -> ModelSignals/15(Mode_GearClutch[1Stim|2Driver|3OpenClutch|4RefGear])  "<Mode_GearClutch[1Stim|2Driver|3OpenClutch|4RefGear]>"
  Bus Selector5/16 -> ModelSignals/16(Gear_Max[0Off|1_n])  "<Gear_Max[0Off|1_n]>"
  Bus Selector5/17 -> ModelSignals/17(State_Engine[0|1|2|3|4])  "<State_Engine[0|1|2|3|4]>"
  Bus Selector5/18 -> ModelSignals/18(State_StartStop[1Off|2NotReady|3Ready|4EngStopped])  "<State_StartStop[1Off|2NotReady|3Ready|4EngStopped]>"
  Bus Selector5/19 -> ModelSignals/19(Sw_Starter[0|1])  "<Sw_Starter[0Off|1On]>"
  Bus Selector5/20 -> ModelSignals/20(CrankAngle_Cyl[aTDC])  "<CrankAngle_Cyl[aTDC]>"
  ModelSignals/1(Out) -> Bus Creator1/1
  Bus Selector5/21 -> ModelSignals/21(Type_Engine_1[0Unkown|1Other|2Otto|3Diesel|4Electric])  "<Type_Engine[0Unkown|1Other|2Otto|3Diesel|4Electric]>"

== system ASM_Traffic_MultiCore/Drivetrain/Interface_Out ==
  note: Drivetrain
  In : Inport
  Animation : Subsystem
  Bus Creator1 : BusCreator  Inputs=3
  Bus Selector2 : BusSelector  OutputSignals=Plant.Drivetrain.Crankshaft.n_Engine[rpm],Plant.Drivetrain.Transmission.OutputSignals.omega_Out_Trm[rad|s],Plant.Drivetrain.Transmission.OutputSignals.Gear[],Plant.Drivetrain.FinalDriveAssembly.i_FinalDrive[],Plant.Drivetrain.FinalDriveAssembly.i_FrontDrive[],Plant.Drivetrain.FinalDriveAssembly.i_RearDrive[],Plant.Drivetrain.FinalDriveAssembly.TrqDistri_Front_Rear[0_1],Plant.Drivetrain.FinalDriveAssembly.Trq_Out_Front_Diff[Nm],Plant.Drivetrain.FinalDriveAssembly.Trq_Shaft[FL;FR;RL;RR][Nm],Plant.Drivetrain.Transmission.OutputSignals.i_unsync_Trm[],Plant.UserInterface.Sw_CrankShaft_Reset[0Disabled|1Enabled],Plant.UserInterface.Mode_Transmission[1Manual|2Automatic],Plant.UserInterface.Mode_Drivetrain[1AWD|2FWD|3RWD|4FF-4WD|5FF],Plant.Drivetrain.Type_Engine_1[0Unkown|1Other|2Otto|3Diesel|4Electric],Plant.Drivetrain.Trq_MeanEff_Engine[Nm],Plant.Drivetrain.Crankshaft.n_Engine[rpm]
  Bus Selector3 : BusSelector  OutputSignals=Plant.Drivetrain.Crankshaft.n_Engine[rpm],Plant.Drivetrain.Transmission.OutputSignals.Gear[]
  Bus Selector4 : BusSelector  OutputSignals=Control.Factor_Trq_Engine_Red[%],Control.Ctrl_Parking_Pawl[0|1]
  Control_ModelSignals : Subsystem
  Plant_ModelSignals : Subsystem
  Trq_BSG[Nm] : Constant  Value=0
  Trq_Engine_2[Nm] : Constant  Value=0
  Type_Engine_2[0Unkown|1Other|2Otto|3Diesel|4Electric] : Constant  Value=0
  n_Engine_2[rpm] : Constant  Value=0
  Out : Outport  VectorParamsAs1DForOutWhenUnconnected=off
  wires:
  n_Engine_2[rpm]/1 -> Plant_ModelSignals/19(n_Engine_2[rpm])
  Bus Selector2/16 -> Plant_ModelSignals/16(n_Engine_1[rpm])  "<n_Engine[rpm]>"
  Bus Selector2/9 -> Plant_ModelSignals/9(Trq_Shaft[FL;FR;RL;RR][Nm])  "<Trq_Shaft[FL;FR;RL;RR][Nm]>"
  Bus Selector2/8 -> Plant_ModelSignals/8(Trq_Out_Front_Diff[Nm])  "<Trq_Out_Front_Diff[Nm]>"
  Bus Selector2/7 -> Plant_ModelSignals/7(TrqDistri_Front_Rear[0_1])  "<TrqDistri_Front_Rear[0_1]>"
  Bus Selector2/6 -> Plant_ModelSignals/6(i_RearDrive[])  "<i_RearDrive[]>"
  Bus Selector2/5 -> Plant_ModelSignals/5(i_FrontDrive[])  "<i_FrontDrive[]>"
  Bus Selector2/2 -> Plant_ModelSignals/2(omega_Out_Trm[rad|s])  "<omega_Out_Trm[rad|s]>"
  Bus Selector3/2 -> Animation/2(Gear[])  "<Gear[]>"
  Bus Selector3/1 -> Animation/1(n_Engine[rpm])  "<n_Engine[rpm]>"
  Bus Selector2/3 -> Plant_ModelSignals/3(Gear[])  "<Gear[]>"
  Bus Selector2/1 -> Plant_ModelSignals/1(n_Engine[rpm])  "<n_Engine[rpm]>"
  Bus Selector2/4 -> Plant_ModelSignals/4(i_FinalDrive[])  "<i_FinalDrive[]>"
  Bus Selector2/10 -> Plant_ModelSignals/10(i_unsync_Trm[])  "<i_unsync_Trm[]>"
  Bus Creator1/1 -> Out/1  "Drivetrain"
  Bus Selector4/2 -> Control_ModelSignals/2(Ctrl_Parking_Pawl[0|1])  "<Ctrl_Parking_Pawl[0|1]>"
  In/1 -> Bus Selector3/1, Bus Selector2/1, Bus Selector4/1
  Bus Selector4/1 -> Control_ModelSignals/1(Factor_Trq_Engine_Red[%])  "<Factor_Trq_Engine_Red[%]>"
  Control_ModelSignals/1(Out) -> Bus Creator1/1
  Trq_BSG[Nm]/1 -> Plant_ModelSignals/20(Trq_BSG[Nm])
  Bus Selector2/11 -> Plant_ModelSignals/11(Sw_CrankShaft_Reset[0Disabled|1Enabled])  "<Sw_CrankShaft_Reset[0Disabled|1Enabled]>"
  Bus Selector2/12 -> Plant_ModelSignals/12(Mode_Transmission[1Manual|2Automatic])  "<Mode_Transmission[1Manual|2Automatic]>"
  Bus Selector2/13 -> Plant_ModelSignals/13(Mode_Drivetrain[1|2|3|4|5])  "<Mode_Drivetrain[1AWD|2FWD|3RWD|4FF-4WD|5FF]>"
  Plant_ModelSignals/1(Out) -> Bus Creator1/2
  Animation/1(Out) -> Bus Creator1/3
  Bus Selector2/14 -> Plant_ModelSignals/14(Type_Engine_1[0Unkown|1Other|2Otto|3Diesel|4Electric])  "<Type_Engine_1[0Unkown|1Other|2Otto|3Diesel|4Electric]>"
  Type_Engine_2[0Unkown|1Other|2Otto|3Diesel|4Electric]/1 -> Plant_ModelSignals/17(Type_Engine_2[0Unkown|1Other|2Otto|3Diesel|4Electric])
  Bus Selector2/15 -> Plant_ModelSignals/15(Trq_Engine_1[Nm])  "<Trq_MeanEff_Engine[Nm]>"
  Trq_Engine_2[Nm]/1 -> Plant_ModelSignals/18(Trq_Engine_2[Nm])

== system ASM_Traffic_MultiCore/Drivetrain/Plant ==
  note: Drivetrain
  Interface_In : Inport
  Control : Inport  Port=2
  drive_trq[Nm] : Inport  Port=3
  Bus Creator : BusCreator  Inputs=2
  Drivetrain : Subsystem
  UserInterface : Subsystem
  Plant : Outport  VectorParamsAs1DForOutWhenUnconnected=off
  wires:
  Interface_In/1 -> Drivetrain/2(Interface_In)
  Control/1 -> Drivetrain/3(Control)
  UserInterface/1(Out) -> Bus Creator/2, Drivetrain/1(UserInterface)
  Drivetrain/1(ASMSignalBus) -> UserInterface/1(In), Bus Creator/1
  Bus Creator/1 -> Plant/1  "Plant"
  drive_trq[Nm]/1 -> Drivetrain/4(drive_trq[Nm])

== system ASM_Traffic_MultiCore/Drivetrain/SignalInterface ==
  In : Inport
  ASMSignalInterface : Subsystem  mask(ASM_SIGNAL_INTERFACE){LabelTextfield=Drivetrain}
      mask prompts: LabelTextfield "Label"
      mask help:
      | The ASMSignalInterface block processes the ASMSignalBus and provides a vector-based interface for each signal (e.g. ModelDesk Plotting).
      |
      | Always push the update button after you have changed the signal bus structure in order to synchronize the signal interface. The update may take a few seconds.
      | A modified model must be reloaded in ModelDesk to keep consistency of ModelDesk and simulation model plot signals. Therefore select ''Update Model'' from the ''Simulation Model'' context menu of the ModelDesk Project Navigator.
      settings: AttributesFormatString=Label: %<LabelTextfield>
      settings: CopyFcn=|
      | try
      |  set_param(gcb,'LinkStatus', 'none')
      | catch
      | end
      mask Help: eval(['asm_modelhelp(gcbh,''tool'',''ASM_Utils_lib'', ''ASMSIGNALINTERFACE'')'])
      mask DialogControl Hint Prompt: For changes of Label first apply change and then push "Update".
      mask DialogControl UpdateButton Prompt: Update
      mask DialogControl UpdateButton Callback: asm_mdld_plot_block_update(bdroot(gcb), 'update', 'current');
      mask DialogControl UpdateAllButton Prompt: Update All
      mask DialogControl UpdateAllButton Callback: asm_mdld_plot_block_update(bdroot(gcb), 'update', 'all');
  Bus Creator : BusCreator  Inputs=2
  Bus Selector Disable Signals : BusSelector  OutputSignals=ExternalModel.Sw_ModelPortBlocks[0Disabled|1Enabled],ExternalModel.Sw_ModelDeskPlottingInterface[0Disabled|1Enabled]
  ExternalOutports : Subsystem  TreatAsAtomicUnit=on
  wires:
  Bus Selector Disable Signals/2 -> ASMSignalInterface/Enable  "<Sw_ModelDeskPlottingInterface[0Disabled|1Enabled]>"
  Bus Selector Disable Signals/1 -> ExternalOutports/Enable  "<Sw_ModelPortBlocks[0Disabled|1Enabled]>"
  In/1 -> Bus Selector Disable Signals/1
  [ASMBUS_Drivetrain_Plant] -> Bus Creator/2, ExternalOutports/1(In1)
  [ASMBUS_Drivetrain_Control] -> Bus Creator/1
  Bus Creator/1 -> ASMSignalInterface/1(ASMSignalBus)

== system ASM_Traffic_MultiCore/ElectricalSystem/Control ==
  note: Electrical System Basic Control
  Interface_In : Inport
  Plant : Inport  Port=2
  SoftECU_ElectricalSystem : Subsystem
  UserInterface : Subsystem
  Control : Outport  VectorParamsAs1DForOutWhenUnconnected=off
  wires:
  SoftECU_ElectricalSystem/2(Out) -> Control/1
  Interface_In/1 -> SoftECU_ElectricalSystem/2(Interface_In)
  SoftECU_ElectricalSystem/1(ASMSignalBus) -> UserInterface/1(In)
  Plant/1 -> SoftECU_ElectricalSystem/3(Plant)
  UserInterface/1(Out) -> SoftECU_ElectricalSystem/1(UserInterface)

== system ASM_Traffic_MultiCore/ElectricalSystem/Interface_In ==
  note: Electrical System Basic
  In : Inport
  Bus Creator : BusCreator  Inputs=1
  Bus Selector : BusSelector  OutputSignals=Environment.Plant.Sw_ModelPortBlocks[0Disabled|1Enabled],Environment.Plant.Sw_ModelDeskPlottingInterface[0Disabled|1Enabled]
  ModelSignals : Subsystem
  Out : Outport  VectorParamsAs1DForOutWhenUnconnected=off
  wires:
  ModelSignals/1(Out) -> Bus Creator/1
  Bus Selector/2 -> ModelSignals/2(Sw_ModelDeskPlottingInterface[0Disabled|1Enabled])  "<Sw_ModelDeskPlottingInterface[0Disabled|1Enabled]>"
  Bus Selector/1 -> ModelSignals/1(Sw_ModelPortBlocks[0Disabled|1Enabled])  "<Sw_ModelPortBlocks[0Disabled|1Enabled]>"
  In/1 -> Bus Selector/1
  Bus Creator/1 -> Out/1

== system ASM_Traffic_MultiCore/ElectricalSystem/Interface_Out ==
  note: Electrical System Basic
  In : Inport
  Bus Creator1 : BusCreator  Inputs=2
  Bus Selector2 : BusSelector  OutputSignals=Control.SOC_Estimated_Max[%],Control.SOC_Estimated_Mean[%]
  Bus Selector7 : BusSelector  OutputSignals=Plant.Battery_LV.V_Bat[V],Plant.Battery_LV.SOC_Bat[%],Plant.Battery_LV.T_Bat[degC],Plant.Battery_HV.V_Bat[V],Plant.Battery_HV.T_Bat[degC],Plant.DCLink.V_DCLink[V]
  Control_ModelSignals : Subsystem
  I_DCDC_LS[A] : Constant  Value=0
  I_DCLink[A] : Constant  Value=0
  Plant_ModelSignals : Subsystem
  State_DCLink[0Off|1On] : Constant
  Sw_DCLink_Reset[0Disabled|1Enabled] : Constant  Value=0
  Out : Outport  VectorParamsAs1DForOutWhenUnconnected=off
  wires:
  I_DCDC_LS[A]/1 -> Plant_ModelSignals/8(I_DCDC_LS[A])
  I_DCLink[A]/1 -> Plant_ModelSignals/7(I_DCLink[A])
  Sw_DCLink_Reset[0Disabled|1Enabled]/1 -> Plant_ModelSignals/10(Sw_DCLink_Reset[0Disabled|1Enabled])
  Bus Selector7/1 -> Plant_ModelSignals/1(V_Bat_LV[V])  "<V_Bat[V]>"
  Bus Selector7/2 -> Plant_ModelSignals/2(SOC_Bat_LV[%])  "<SOC_Bat[%]>"
  Bus Selector7/3 -> Plant_ModelSignals/3(T_Bat_LV[degC])  "<T_Bat[degC]>"
  Bus Selector7/4 -> Plant_ModelSignals/4(V_Bat_HV[V])  "<V_Bat[V]>"
  Bus Selector7/5 -> Plant_ModelSignals/5(T_Bat_HV[degC])  "<T_Bat[degC]>"
  Bus Selector7/6 -> Plant_ModelSignals/6(V_DCLink[V])  "<V_DCLink[V]>"
  State_DCLink[0Off|1On]/1 -> Plant_ModelSignals/9(State_DCLink[0Off|1On])
  Bus Creator1/1 -> Out/1  "ElectricalSystem"
  Bus Selector2/2 -> Control_ModelSignals/2(SOC_Estimated_Mean[%])  "<SOC_Estimated_Mean[%]>"
  In/1 -> Bus Selector7/1, Bus Selector2/1
  Control_ModelSignals/1(Out) -> Bus Creator1/1
  Bus Selector2/1 -> Control_ModelSignals/1(SOC_Estimated_Max[%])  "<SOC_Estimated_Max[%]>"
  Plant_ModelSignals/1(Out) -> Bus Creator1/2

== system ASM_Traffic_MultiCore/ElectricalSystem/Plant ==
  note: Electrical System Basic
  Interface_In : Inport
  Control : Inport  Port=2
  ElectricalSystemBasic : Subsystem
  UserInterface : Subsystem
  Plant : Outport  VectorParamsAs1DForOutWhenUnconnected=off
  wires:
  ElectricalSystemBasic/1(ASMSignalBus) -> Plant/1, UserInterface/1(In)
  Interface_In/1 -> ElectricalSystemBasic/2(Interface_In)
  UserInterface/1(Out) -> ElectricalSystemBasic/1(UserInterface)
  Control/1 -> ElectricalSystemBasic/3(Control)
